simulink model "current_loop_noAW"  (R2025b)
settings: Solver=VariableStepAuto  StartTime=0.0  StopTime=2  RelTol=1e-3
values from neighbouring files (symbols this model uses):
  p = params()    [test_fdi_attack_types.m]    (also in test_fdi_control_attack.m; test_fdi_dp.m; test_fdi_dp_control.m; test_fdi_dp_scenarios.m)
libraries: slpidlib x1
settings Model: Creator=Dawid  LastModifiedBy=Dawid

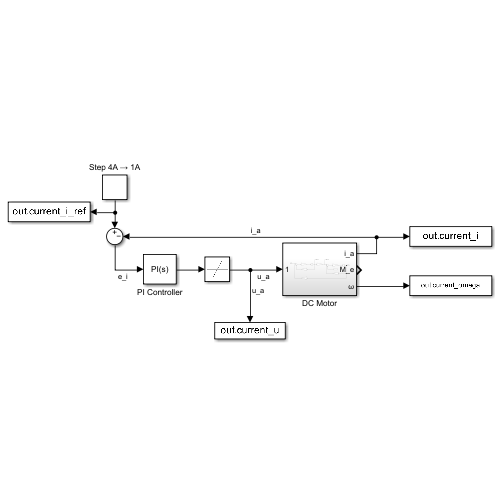
[thumbnail: Simulink's stored preview of the top-level diagram]
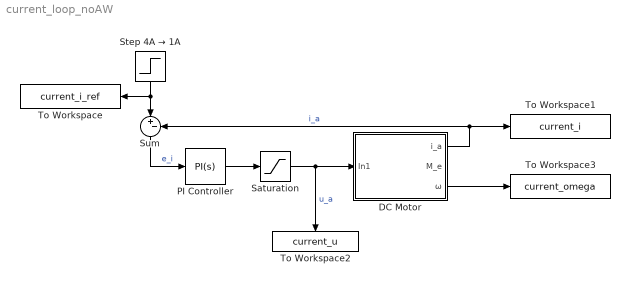
== system current_loop_noAW ==
  DC Motor : Subsystem
  PI Controller : slpidlib/PID Controller  Controller=PI  Form=Parallel  TimeDomain=Continuous-time  UseExternalTs=off  SampleTime=-1  IntegratorMethod=Forward Euler  FilterMethod=Forward Euler  ControllerParametersSource=internal  P=p.control.current.Kp  I=p.control.current.Ki  UseKiTs=off  D=0  UseExternalDerivativeSource=off  N=100  UseFilter=on  TunerSelectOption=Transfer Function Based (PID Tuner App)  InitialConditionSource=internal  InitialConditionForIntegrator=0  InitialConditionForFilter=0  DifferentiatorICPrevScaledInput=0  ExternalReset=none  TrackingMode=off  Kt=1  LimitOutput=off  SatLimitsSource=internal  UpperSaturationLimit=p.limits.Umax  LowerSaturationLimit=p.limits.Umin  LinearizeAsGain=on  AntiWindupMode=back-calculation  Kb=p.control.current.Kb  LimitIntegrator=off  UpperIntegratorSaturationLimit=inf  LowerIntegratorSaturationLimit=-inf  POutMin=[]  POutMax=[]  IOutMin=[]  IOutMax=[]  DOutMin=[]  DOutMax=[]  NOutMin=[]  NOutMax=[]  SumOutMin=[]  SumOutMax=[]  SaturationOutMin=[]  SaturationOutMax=[]  PParamMin=[]  PParamMax=[]  IParamMin=[]  IParamMax=[]  DParamMin=[]  DParamMax=[]  NParamMin=[]  NParamMax=[]  KbParamMin=[]  KbParamMax=[]  KtParamMin=[]  KtParamMax=[]  KbOutMin=[]  KbOutMax=[]  KtOutMin=[]  KtOutMax=[]  IntegratorOutMin=[]  IntegratorOutMax=[]  FilterOutMin=[]  FilterOutMax=[]  SumI1OutMin=[]  SumI1OutMax=[]  SumI2OutMin=[]  SumI2OutMax=[]  SumI3OutMin=[]  SumI3OutMax=[]  SumI4OutMin=[]  SumI4OutMax=[]  SumDOutMin=[]  SumDOutMax=[]  DifferentiatorOutMin=[]  DifferentiatorOutMax=[]  FilterDiffOutCoefMin=[]  FilterDiffOutCoefMax=[]  ReciprocalOutMin=[]  ReciprocalOutMax=[]  SumDenOutMin=[]  SumDenOutMax=[]  SumNumOutMin=[]  SumNumOutMax=[]  DivideOutMin=[]  DivideOutMax=[]  UdiffTsProdOutMin=[]  UdiffTsProdOutMax=[]  NTsProdOutMin=[]  NTsProdOutMax=[]  UintegralTsProdOutMin=[]  UintegralTsProdOutMax=[]  UngainTsProdOutMin=[]  UngainTsProdOutMax=[]  ClampingZeroOutDataTypeStr=Inherit: Inherit via back propagation  ClampingZeroOutMin=[]  ClampingZeroOutMax=[]  FilterDenConstantOutDataTypeStr=Inherit: Inherit via back propagation  FilterDenConstantOutMin=[]  FilterDenConstantOutMax=[]  PCopyOutDataTypeStr=Inherit: Inherit via back propagation  PCopyOutMin=[]  PCopyOutMax=[]  NCopyOutDataTypeStr=Inherit: Inherit via back propagation  NCopyOutMin=[]  NCopyOutMax=[]  IntegratorContinuousStateAttributes=''  IntegratorStateMustResolveToSignalObject=off  IntegratorRTWStateStorageClass=Auto  FilterContinuousStateAttributes=''  FilterStateMustResolveToSignalObject=off  FilterRTWStateStorageClass=Auto  ParallelPVariant=InternalParameters  IdealPVariant=Disabled  IVariant=InternalParameters  DVariant=Disabled  IntegratorVariant=Continuous  SatVariant=Disabled  AWVariant=Passthrough  PCopyVariant=Disabled  TRVariant=Disabled  FdbkBlocksVariant=Forward  IdealPFdbkVariant=Disabled  SatFdbkVariant=Disabled  DerivativeFilterVariant=Disabled  NVariant=Disabled  NCopyVariant=Disabled_SignalSpec  FilterICVariant=Disabled  IntegratorICVariant=InternalICs  ExternalResetVariant=Disabled  TRSumVariant=Passthrough  SumFdbkVariant=Disabled  SumVariant=Sum_PI  TsampFilterVariant=InternalTs  TsampNgainVariant=Passthrough  TsampIntegralVariant=Disabled_SignalSpec  ExternalSaturationOutDataTypeStr=Inherit: Same as second input  DerivativeSourceVariant=Disabled  PreIntVariant=InternalPreInt
  Saturation : Saturate  UpperLimit=p.limits.Umax  LowerLimit=p.limits.Umin
  Step 4A → 1A : Step  Time=0.1  Before=4  SampleTime=0
  Sum : Sum  Inputs=|+-
  To Workspace : ToWorkspace  VariableName=current_i_ref  SaveFormat=Timeseries  SampleTime=-1
  To Workspace1 : ToWorkspace  VariableName=current_i  SaveFormat=Timeseries  SampleTime=-1
  To Workspace2 : ToWorkspace  VariableName=current_u  SaveFormat=Timeseries  SampleTime=-1
  To Workspace3 : ToWorkspace  VariableName=current_omega  SaveFormat=Timeseries  SampleTime=-1
  wires:
  Step 4A → 1A/1 -> Sum/1, To Workspace/1
  Sum/1 -> PI Controller/1  "e_i"
  PI Controller/1 -> Saturation/1
  DC Motor/1(i_a) -> Sum/2, To Workspace1/1  "i_a"
  DC Motor/3(ω) -> To Workspace3/1
  Saturation/1 -> DC Motor/1(In1), To Workspace2/1  "u_a"

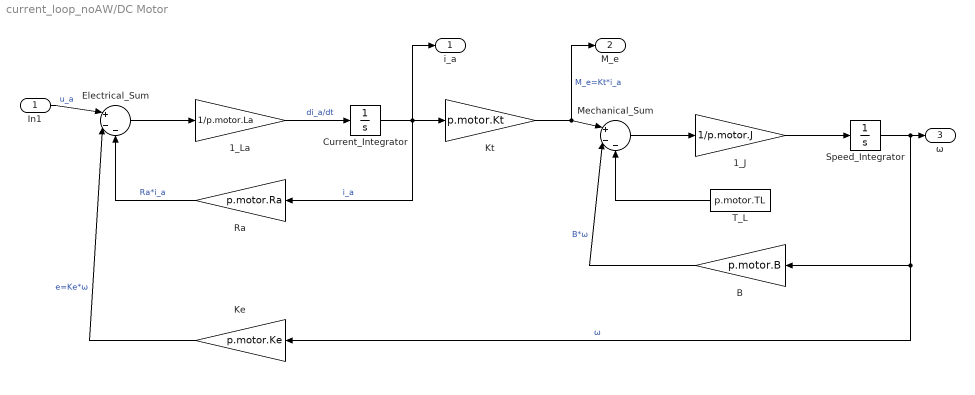
== system current_loop_noAW/DC Motor ==
  In1 : Inport
  1_J : Gain  Gain=1/p.motor.J
  1_La : Gain  Gain=1/p.motor.La
  B : Gain  Gain=p.motor.B
  Current_Integrator : Integrator  InitialCondition=p.initial.i_a
  Electrical_Sum : Sum  Inputs=|+--
  Ke : Gain  Gain=p.motor.Ke
  Kt : Gain  Gain=p.motor.Kt
  Mechanical_Sum : Sum  Inputs=|+--
  Ra : Gain  Gain=p.motor.Ra
  Speed_Integrator : Integrator  InitialCondition=p.initial.omega
  T_L : Constant  Value=p.motor.TL
  i_a : Outport
  M_e : Outport  Port=2
  ω : Outport  Port=3
  wires:
  Speed_Integrator/1 -> B/1, Ke/1, ω/1  "ω"
  Current_Integrator/1 -> i_a/1, Kt/1, Ra/1  "i_a"
  T_L/1 -> Mechanical_Sum/3
  Kt/1 -> M_e/1, Mechanical_Sum/1  "M_e=Kt*i_a"
  1_La/1 -> Current_Integrator/1  "di_a/dt"
  Electrical_Sum/1 -> 1_La/1
  Ra/1 -> Electrical_Sum/3  "Ra*i_a"
  Mechanical_Sum/1 -> 1_J/1
  1_J/1 -> Speed_Integrator/1
  B/1 -> Mechanical_Sum/2  "B*ω"
  Ke/1 -> Electrical_Sum/2  "e=Ke*ω"
  In1/1 -> Electrical_Sum/1  "u_a"
